simulink model "mpc_ttype_psm"  (R2026a)
settings: Solver=ode23tb  StopTime=param.sim.simlength  FixedStep=param.glb_time.tc  MaxStep=param.glb_time.tc
values from neighbouring files (symbols this model uses):
  param = struct()    [init_model.m]
libraries: fl_lib x25, nesl_utility x12, cstblocks_lti x6, lithium_ion_battery x1, dclink_for_three_levels x1, three_phase_three_level_ttype_inverter_ideal_switch_based_model x1, single_phase_pwm_modulator x1, threephase_inductor_lib x1, simple_flexible_shaft x1, permanent_magnet_synchronous_machine x1
(part 1 of 4)
settings Model: SimulationMode=accelerator  Creator=dbagn  LastModifiedBy=dbagn
settings SolverCC: NumberNewtonIterations=3.0  ZeroCrossControl=DisableAll  SolverResetMethod=Robust
settings SFSimCC: CustomCodeUndefinedFunction=ThrowError  DefaultCustomCodeDeterministicFunctions=All
settings SFSimCC: SimCustomHeaderCode=|
  | #include "rpi.h"
  | #include "mavgflt.h"
  | #include "mavgflt_simulink.h"
  | #include "mavgflts.h"
  | #include "mavgflts_simulink.h"
  | #include "dsmavgflt.h"
  | #include "dsmavgflt_simulink.h"
  | #include "bemf_obsv.h"
  | #include "bemf_obsv_simulink.h"
  | #include "bemf_obsv_load_est.h"
  | #include "bemf_obsv_load_est_simulink.h"
  | #include "dqvector_pi.h"
  | #include "dqvector_pi_simulink.h"
  | #include "sv_pwm_simulink.h"
  | #include "sv_pwm.h"
  | #include "first_harmonic_tracker.h"
  | #include "first_harmonic_tracker_simulink.h"
  | #include "dqpll_thyr.h"
  | #include "dqpll_thyr_simulink.h"
  | #include "dqpll_grid.h"
  | #include "dqpll_grid_simulink.h"
settings SFSimCC: SimUserSources=|
  | "rpi.c"
  | "mavgflt_simulink.c"
  | "mavgflt.c"
  | "mavgflts_simulink.c"
  | "mavgflts.c"
  | "dsmavgflt_simulink.c"
  | "dsmavgflt.c"
  | "bemf_obsv_simulink.c"
  | "bemf_obsv.c"
  | "bemf_obsv_load_est_simulink.c"
  | "bemf_obsv_load_est.c"
  | "dqvector_pi.c"
  | "dqvector_pi_simulink.c"
  | "sv_pwm_simulink.c"
  | "sv_pwm.c"
  | "first_harmonic_tracker_simulink.c"
  | "first_harmonic_tracker.c"
  | "dqpll_thyr_simulink.c"
  | "dqpll_thyr.c"
  | "dqpll_grid_simulink.c"
  | "dqpll_grid.c"
settings SFSimCC: SimUserIncludeDirs=|
  | include
  | src
settings SimscapeCC: SimscapeNominalValues="[{\"value\":\"1\",\"unit\":\"A\"},{\"value\":\"1\",\"unit\":\"bar\"},{\"value\":\"1\",\"unit\":\"cm^2\"},{\"value\":\"1\",\"unit\":\"cm^3/s\"},{\"value\":\"1\",\"unit\":\"kJ/kg\"},{\"value\":\"1\",\"unit\":\"kW\"},{\"value\":\"1\",\"unit\":\"l\"},{\"value\":\"1\",\"unit\":\"N\"},{\"value\":\"1\",\"unit\":\"N*m\"},{\"value\":\"1\",\"unit\":\"V\"}]"  SimscapeLogType=none  SimscapeLogDataHistory=5000.0

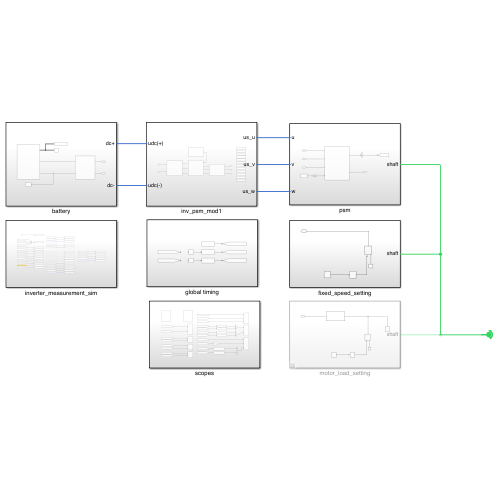
[thumbnail: Simulink's stored preview of the top-level diagram]
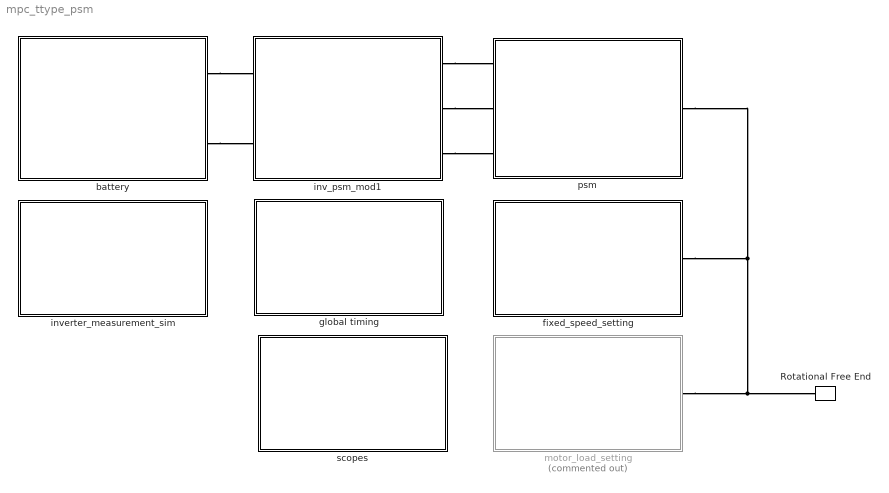
== system mpc_ttype_psm ==
  Rotational Free End : fl_lib/Mechanical/Rotational Elements/Rotational Free End  w_specify=off  w_priority=None  w=0 rad/s  w_nominal_specify=off  w_nominal_value=1  w_nominal_unit=rad/s
  battery : Subsystem
  fixed_speed_setting : Subsystem
  global timing : Subsystem
  inv_psm_mod1 : Subsystem
  inverter_measurement_sim : Subsystem
  motor_load_setting : Subsystem  Commented=on
  psm : Subsystem
  scopes : Subsystem
  connections:
  psm/RConn1 -- fixed_speed_setting/LConn1 -- motor_load_setting/LConn1 -- Rotational Free End/LConn1
  inv_psm_mod1/RConn2 -- psm/LConn2
  inv_psm_mod1/RConn1 -- psm/LConn1
  inv_psm_mod1/RConn3 -- psm/LConn3
  battery/RConn1 -- inv_psm_mod1/LConn1
  battery/RConn2 -- inv_psm_mod1/LConn2

== system mpc_ttype_psm/battery ==
  Solver Configuration : nesl_utility/Solver Configuration  PhysicalDomain=network_engine_domain  SubClassName=solver  LeftPortType=input  RightPortType=generic  Tones=[]  Harmonics=[]  SimulateNoise=off  Profile=off  UseLocalSampling=off  EnableSwitchedLinearOptims=on  FrequencyDomain=off  UseCCode=off  RelTol=0.001  AbsTol=0.001  MinStep=1e-09  ToWorkspace=off  RevertToSquareIcSolve=off  NumHomotopyIterations=100  PhasorMode=off  PhasorModeNumHarmonics=1  ConsistencySolver=NEWTON_FTOL  CanonicalOrdering=UNORDERED  OptimizeIntermediates=UNOPTIMIZED  IndexReductionMethod=DerivativeReplacement  DoDC=on  ResidualTolerance=1e-09  ConsistencyTolSource=GLOBAL  ConsistencyAbsTol=0.001  ConsistencyRelTol=0.001  ConsistencyTolFactor=0.001  UseLocalSolver=on  LocalSolverChoice=NE_BACKWARD_EULER_ADVANCER  ResolveIndetEquations=on  FunctionEvalNumThread=1  LocalSolverSampleTime=param.glb_time.tc  DoFixedCost=on  MaxNonlinIter=param.sim.nonlinear_iterations  MaxModeIter=2  ComputeImpulses=off  ImpulseIterations=2  LinearAlgebra=auto  LinearAlgebraNumThread=0  EquationFormulation=NE_TIME_EF  DelaysMemoryBudget=1024  AutomaticFiltering=on  FilteringTimeConstant=0.001  PartitionStorageMethod=AS_NEEDED  PartitionMemoryBudget=1024  PartitionMethod=ROBUST  MultibodyUseLocalSolver=off  MultibodyLocalSolverChoice=ODE1  MultibodyLocalSolverSampleTime=0.001
  To Workspace14 : ToWorkspace  VariableName=battery_data  SampleTime=param.glb_time.tc
      settings: MaxDataPoints=param.glb_time.Nc
  lithium ion battery : Scope
      settings: ActiveDisplayYMinimum=-146.3940131322023  ActiveDisplayYMaximum=1008.7733008785125  DataLoggingVariableName=ScopeData3
  lithium_ion_battery : lithium_ion_battery/lithium_ion_battery  Q=param.battery.pack_1.Q  number_of_cells=param.battery.pack_1.number_of_cells  E_1=param.battery.pack_1.E_1  E0=param.battery.pack_1.E0  E1=param.battery.pack_1.E1  E2=param.battery.pack_1.E2  E3=param.battery.pack_1.E3  Elog=param.battery.pack_1.Elog  R0=param.battery.pack_1.R0  R1=param.battery.pack_1.R1  C1=param.battery.pack_1.C1  M=param.battery.pack_1.M  alpha=param.battery.pack_1.alpha  soc_init=param.battery.pack_1.soc_init  ts_battery=param.glb_time.ts_dab  q1Kalman=param.battery.pack_1.q1Kalman  q2Kalman=param.battery.pack_1.q2Kalman  q3Kalman=param.battery.pack_1.q3Kalman  rKalman=param.battery.pack_1.rKalman  tc=param.glb_time.tc  enable_white_noise_m=0
  single_phase_ui_measure : Subsystem
  dc+ : PMIOPort  Side=Right
  dc- : PMIOPort  Port=2  Side=Right
  wires:
  lithium_ion_battery/1 -> To Workspace14/1, lithium ion battery/1
  connections:
  single_phase_ui_measure/LConn2 -- Solver Configuration/RConn1 -- lithium_ion_battery/RConn2
  single_phase_ui_measure/RConn1 -- dc+/RConn1
  lithium_ion_battery/RConn1 -- single_phase_ui_measure/LConn1
  dc-/RConn1 -- single_phase_ui_measure/RConn2

== system mpc_ttype_psm/fixed_speed_setting ==
  Ideal Angular Velocity Source : fl_lib/Mechanical/Mechanical Sources/Ideal Angular Velocity Source
  Mechanical Rotational Reference : fl_lib/Mechanical/Rotational Elements/Mechanical Rotational Reference
  PS Step1 : fl_lib/Physical Signals/Sources/PS Step  step_time=0.025 s  initial_value=0 rpm  final_value=param.load.rpm_sim rpm
  PS Transfer Function : fl_lib/Physical Signals/Linear Operators/PS Transfer Function  transfer_function_type=foundation.enum.transfer_function_type.lag  T=0.1 s  T1=2 s  T2=1 s  reset_method=foundation.enum.IntegratorResetSpec.None  initial_condition_spec=foundation.enum.IntegratorICSpec.Internal  y0=0 rpm
  shaft : PMIOPort  Side=Left
  connections:
  Mechanical Rotational Reference/LConn1 -- Ideal Angular Velocity Source/RConn2
  PS Step1/RConn1 -- PS Transfer Function/LConn1
  PS Transfer Function/RConn1 -- Ideal Angular Velocity Source/RConn1
  Ideal Angular Velocity Source/LConn1 -- shaft/RConn1

== system mpc_ttype_psm/global timing ==
  From9 : From  Commented=on  GotoTag=local_time_corr_afe1
  Unit Delay : UnitDelay  SampleTime=param.glb_time.tc
  Unit Delay1 : UnitDelay  SampleTime=param.glb_time.tc
  time_afe1 : Subsystem  mask{k=param.afe.behav.time_gain_module_1}
      mask prompts: k "Time Gain"
      mask Display:
      | disp('time-gen');
      | port_label('input', 1, 'crt');
      | port_label('output', 1, 'tout');
  time_afe3 : Subsystem  mask{k=1}
      mask prompts: k "Time Gain"
      mask Display:
      | disp('time-gen');
      | port_label('output', 1, 'tout');
  time_inv1 : Subsystem  mask{k=param.inv.behav.time_gain_module_2}
      mask prompts: k "Time Gain"
      mask Display:
      | disp('time-gen');
      | port_label('input', 1, 'crt');
      | port_label('output', 1, 'tout');
  tag scope: time_afe_module_1=global, time_inv_module_1=global, time_master=global
  wires:
  time_afe1/1(Out1) -> [time_afe_module_1]
  time_inv1/1(Out1) -> [time_inv_module_1]
  time_afe3/1(Out1) -> [time_master]
  Unit Delay/1 -> time_afe1/1(correction_time)
  Unit Delay1/1 -> time_inv1/1(correction_time)

== system mpc_ttype_psm/inv_psm_mod1 ==
  Goto Tag Visibility : GotoTagVisibility  GotoTag=vdc_pu
  Goto Tag Visibility1 : GotoTagVisibility  GotoTag=udc
  Goto Tag Visibility10 : GotoTagVisibility  GotoTag=udc1_pu
  Goto Tag Visibility11 : GotoTagVisibility  GotoTag=udc2_pu
  Goto Tag Visibility2 : GotoTagVisibility  GotoTag=udc1
  Goto Tag Visibility3 : GotoTagVisibility  GotoTag=udc2
  Goto Tag Visibility4 : GotoTagVisibility  GotoTag=np_current
  Goto Tag Visibility5 : GotoTagVisibility  GotoTag=udc_p_gnd
  Goto Tag Visibility6 : GotoTagVisibility  GotoTag=udc_n_gnd
  Goto Tag Visibility7 : GotoTagVisibility  GotoTag=udc_centertap_gnd
  Goto Tag Visibility8 : GotoTagVisibility  GotoTag=Cdc1_current
  Goto Tag Visibility9 : GotoTagVisibility  GotoTag=Cdc2_current
  dclink : Subsystem
  inverter : Subsystem
  inverter_ctrl : Subsystem
  inverter_output_filter : Subsystem
  us_u : PMIOPort  Side=Right
  us_v : PMIOPort  Port=2  Side=Right
  us_w : PMIOPort  Port=3  Side=Right
  udc(+) : PMIOPort  Port=4  Side=Left
  udc(-) : PMIOPort  Port=5  Side=Left
  wires:
  inverter_ctrl/1(cmd_gates) -> inverter/1(gate_cmds_uvw)
  connections:
  inverter_output_filter/LConn2 -- us_v/RConn1
  inverter_output_filter/LConn3 -- us_w/RConn1
  inverter_output_filter/LConn1 -- us_u/RConn1
  dclink/LConn1 -- udc(+)/RConn1
  dclink/LConn2 -- udc(-)/RConn1
  inverter/RConn2 -- dclink/RConn2
  inverter/RConn1 -- dclink/RConn1
  inverter/RConn3 -- dclink/RConn3
  inverter_output_filter/RConn3 -- inverter/LConn3
  inverter_output_filter/RConn2 -- inverter/LConn2
  inverter_output_filter/RConn1 -- inverter/LConn1

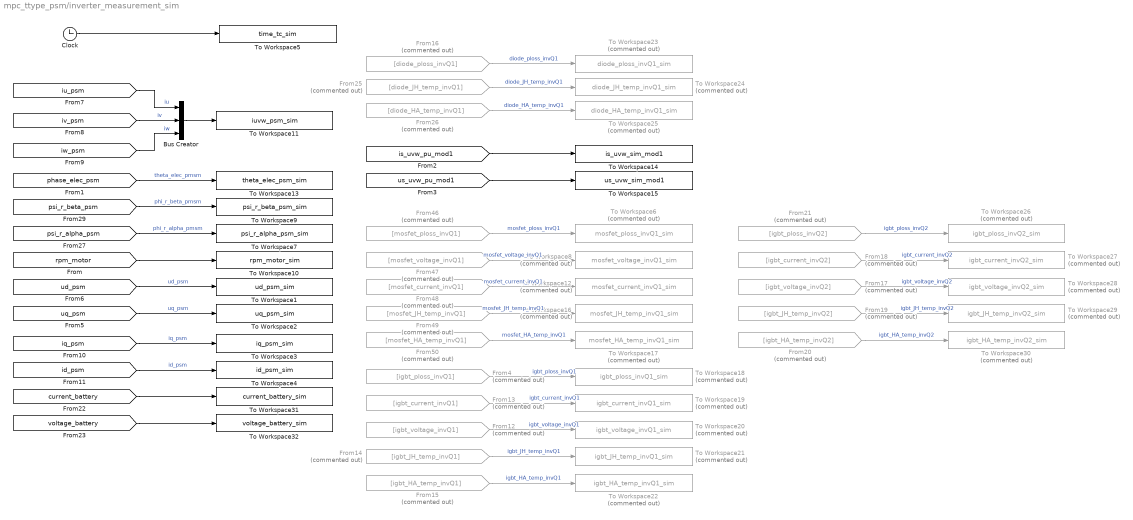
== system mpc_ttype_psm/inverter_measurement_sim ==
  Bus Creator : BusCreator  Inputs=3
  Clock : Clock
  From12 : From  Commented=on  GotoTag=igbt_voltage_invQ1
  From13 : From  Commented=on  GotoTag=igbt_current_invQ1
  From14 : From  Commented=on  GotoTag=igbt_JH_temp_invQ1
  From15 : From  Commented=on  GotoTag=igbt_HA_temp_invQ1
  From16 : From  Commented=on  GotoTag=diode_ploss_invQ1
  From17 : From  Commented=on  GotoTag=igbt_voltage_invQ2
  From18 : From  Commented=on  GotoTag=igbt_current_invQ2
  From19 : From  Commented=on  GotoTag=igbt_JH_temp_invQ2
  From20 : From  Commented=on  GotoTag=igbt_HA_temp_invQ2
  From21 : From  Commented=on  GotoTag=igbt_ploss_invQ2
  From25 : From  Commented=on  GotoTag=diode_JH_temp_invQ1
  From26 : From  Commented=on  GotoTag=diode_HA_temp_invQ1
  From4 : From  Commented=on  GotoTag=igbt_ploss_invQ1
  From46 : From  Commented=on  GotoTag=mosfet_ploss_invQ1
  From47 : From  Commented=on  GotoTag=mosfet_voltage_invQ1
  From48 : From  Commented=on  GotoTag=mosfet_current_invQ1
  From49 : From  Commented=on  GotoTag=mosfet_JH_temp_invQ1
  From50 : From  Commented=on  GotoTag=mosfet_HA_temp_invQ1
  To Workspace1 : ToWorkspace  VariableName=ud_psm_sim  SampleTime=param.glb_time.tc
      settings: MaxDataPoints=param.glb_time.Nc  Save2DSignal=2-D array (concatenate along first dimension)
  To Workspace10 : ToWorkspace  VariableName=rpm_motor_sim  SampleTime=param.glb_time.tc
      settings: MaxDataPoints=param.glb_time.Nc  Save2DSignal=2-D array (concatenate along first dimension)
  To Workspace11 : ToWorkspace  VariableName=iuvw_psm_sim  SampleTime=param.glb_time.tc
      settings: MaxDataPoints=param.glb_time.Nc  Save2DSignal=2-D array (concatenate along first dimension)
  To Workspace12 : ToWorkspace  Commented=on  VariableName=mosfet_current_invQ1_sim  SampleTime=param.glb_time.tc
      settings: MaxDataPoints=param.glb_time.Nc  Save2DSignal=2-D array (concatenate along first dimension)
  To Workspace13 : ToWorkspace  VariableName=theta_elec_psm_sim  SampleTime=param.glb_time.tc
      settings: MaxDataPoints=param.glb_time.Nc  Save2DSignal=2-D array (concatenate along first dimension)
  To Workspace14 : ToWorkspace  VariableName=is_uvw_sim_mod1  SampleTime=param.glb_time.tc
      settings: MaxDataPoints=param.glb_time.Nc  Save2DSignal=2-D array (concatenate along first dimension)
  To Workspace15 : ToWorkspace  VariableName=us_uvw_sim_mod1  SampleTime=param.glb_time.tc
      settings: MaxDataPoints=param.glb_time.Nc  Save2DSignal=2-D array (concatenate along first dimension)
  To Workspace16 : ToWorkspace  Commented=on  VariableName=mosfet_JH_temp_invQ1_sim  SampleTime=param.glb_time.tc
      settings: MaxDataPoints=param.glb_time.Nc  Save2DSignal=2-D array (concatenate along first dimension)
  To Workspace17 : ToWorkspace  Commented=on  VariableName=mosfet_HA_temp_invQ1_sim  SampleTime=param.glb_time.tc
      settings: MaxDataPoints=param.glb_time.Nc  Save2DSignal=2-D array (concatenate along first dimension)
  To Workspace18 : ToWorkspace  Commented=on  VariableName=igbt_ploss_invQ1_sim  SampleTime=param.glb_time.tc
      settings: MaxDataPoints=param.glb_time.Nc  Save2DSignal=2-D array (concatenate along first dimension)
  To Workspace19 : ToWorkspace  Commented=on  VariableName=igbt_current_invQ1_sim  SampleTime=param.glb_time.tc
      settings: MaxDataPoints=param.glb_time.Nc  Save2DSignal=2-D array (concatenate along first dimension)
  To Workspace2 : ToWorkspace  VariableName=uq_psm_sim  SampleTime=param.glb_time.tc
      settings: MaxDataPoints=param.glb_time.Nc  Save2DSignal=2-D array (concatenate along first dimension)
  To Workspace20 : ToWorkspace  Commented=on  VariableName=igbt_voltage_invQ1_sim  SampleTime=param.glb_time.tc
      settings: MaxDataPoints=param.glb_time.Nc  Save2DSignal=2-D array (concatenate along first dimension)
  To Workspace21 : ToWorkspace  Commented=on  VariableName=igbt_JH_temp_invQ1_sim  SampleTime=param.glb_time.tc
      settings: MaxDataPoints=param.glb_time.Nc  Save2DSignal=2-D array (concatenate along first dimension)
  To Workspace22 : ToWorkspace  Commented=on  VariableName=igbt_HA_temp_invQ1_sim  SampleTime=param.glb_time.tc
      settings: MaxDataPoints=param.glb_time.Nc  Save2DSignal=2-D array (concatenate along first dimension)
  To Workspace23 : ToWorkspace  Commented=on  VariableName=diode_ploss_invQ1_sim  SampleTime=param.glb_time.tc
      settings: MaxDataPoints=param.glb_time.Nc
  To Workspace24 : ToWorkspace  Commented=on  VariableName=diode_JH_temp_invQ1_sim  SampleTime=param.glb_time.tc
      settings: MaxDataPoints=param.glb_time.Nc
  To Workspace25 : ToWorkspace  Commented=on  VariableName=diode_HA_temp_invQ1_sim  SampleTime=param.glb_time.tc
      settings: MaxDataPoints=param.glb_time.Nc
  To Workspace26 : ToWorkspace  Commented=on  VariableName=igbt_ploss_invQ2_sim  SampleTime=param.glb_time.tc
      settings: MaxDataPoints=param.glb_time.Nc  Save2DSignal=2-D array (concatenate along first dimension)
  To Workspace27 : ToWorkspace  Commented=on  VariableName=igbt_current_invQ2_sim  SampleTime=param.glb_time.tc
      settings: MaxDataPoints=param.glb_time.Nc  Save2DSignal=2-D array (concatenate along first dimension)
  To Workspace28 : ToWorkspace  Commented=on  VariableName=igbt_voltage_invQ2_sim  SampleTime=param.glb_time.tc
      settings: MaxDataPoints=param.glb_time.Nc  Save2DSignal=2-D array (concatenate along first dimension)
  To Workspace29 : ToWorkspace  Commented=on  VariableName=igbt_JH_temp_invQ2_sim  SampleTime=param.glb_time.tc
      settings: MaxDataPoints=param.glb_time.Nc  Save2DSignal=2-D array (concatenate along first dimension)
  To Workspace3 : ToWorkspace  VariableName=iq_psm_sim  SampleTime=param.glb_time.tc
      settings: MaxDataPoints=param.glb_time.Nc  Save2DSignal=2-D array (concatenate along first dimension)
  To Workspace30 : ToWorkspace  Commented=on  VariableName=igbt_HA_temp_invQ2_sim  SampleTime=param.glb_time.tc
      settings: MaxDataPoints=param.glb_time.Nc  Save2DSignal=2-D array (concatenate along first dimension)
  To Workspace31 : ToWorkspace  VariableName=current_battery_sim  SampleTime=param.glb_time.tc
      settings: MaxDataPoints=param.glb_time.Nc  Save2DSignal=2-D array (concatenate along first dimension)
  To Workspace32 : ToWorkspace  VariableName=voltage_battery_sim  SampleTime=param.glb_time.tc
      settings: MaxDataPoints=param.glb_time.Nc  Save2DSignal=2-D array (concatenate along first dimension)
  To Workspace4 : ToWorkspace  VariableName=id_psm_sim  SampleTime=param.glb_time.tc
      settings: MaxDataPoints=param.glb_time.Nc  Save2DSignal=2-D array (concatenate along first dimension)
  To Workspace5 : ToWorkspace  VariableName=time_tc_sim  SampleTime=param.glb_time.tc
      settings: MaxDataPoints=param.glb_time.Nc  Save2DSignal=2-D array (concatenate along first dimension)
  To Workspace6 : ToWorkspace  Commented=on  VariableName=mosfet_ploss_invQ1_sim  SampleTime=param.glb_time.tc
      settings: MaxDataPoints=param.glb_time.Nc  Save2DSignal=2-D array (concatenate along first dimension)
  To Workspace7 : ToWorkspace  VariableName=psi_r_alpha_psm_sim  SampleTime=param.glb_time.tc
      settings: MaxDataPoints=param.glb_time.Nc  Save2DSignal=2-D array (concatenate along first dimension)
  To Workspace8 : ToWorkspace  Commented=on  VariableName=mosfet_voltage_invQ1_sim  SampleTime=param.glb_time.tc
      settings: MaxDataPoints=param.glb_time.Nc  Save2DSignal=2-D array (concatenate along first dimension)
  To Workspace9 : ToWorkspace  VariableName=psi_r_beta_psm_sim  SampleTime=param.glb_time.tc
      settings: MaxDataPoints=param.glb_time.Nc  Save2DSignal=2-D array (concatenate along first dimension)
  wires:
  [psi_r_alpha_psm] -> To Workspace7/1  "phi_r_alpha_pmsm"
  [psi_r_beta_psm] -> To Workspace9/1  "phi_r_beta_pmsm"
  [rpm_motor] -> To Workspace10/1
  [iv_psm] -> Bus Creator/2  "iv"
  [iw_psm] -> Bus Creator/3  "iw"
  [iu_psm] -> Bus Creator/1  "iu"
  Bus Creator/1 -> To Workspace11/1
  [phase_elec_psm] -> To Workspace13/1  "theta_elec_pmsm"
  [ud_psm] -> To Workspace1/1  "ud_psm"
  [uq_psm] -> To Workspace2/1  "uq_psm"
  [iq_psm] -> To Workspace3/1  "iq_psm"
  [id_psm] -> To Workspace4/1  "id_psm"
  Clock/1 -> To Workspace5/1
  From46/1 -> To Workspace6/1  "mosfet_ploss_invQ1"
  From49/1 -> To Workspace16/1  "mosfet_JH_temp_invQ1"
  From50/1 -> To Workspace17/1  "mosfet_HA_temp_invQ1"
  [is_uvw_pu_mod1] -> To Workspace14/1
  [us_uvw_pu_mod1] -> To Workspace15/1
  From47/1 -> To Workspace8/1  "mosfet_voltage_invQ1"
  From48/1 -> To Workspace12/1  "mosfet_current_invQ1"
  From4/1 -> To Workspace18/1  "igbt_ploss_invQ1"
  From13/1 -> To Workspace19/1  "igbt_current_invQ1"
  From12/1 -> To Workspace20/1  "igbt_voltage_invQ1"
  From14/1 -> To Workspace21/1  "igbt_JH_temp_invQ1"
  From15/1 -> To Workspace22/1  "igbt_HA_temp_invQ1"
  From16/1 -> To Workspace23/1  "diode_ploss_invQ1"
  From25/1 -> To Workspace24/1  "diode_JH_temp_invQ1"
  From26/1 -> To Workspace25/1  "diode_HA_temp_invQ1"
  From20/1 -> To Workspace30/1  "igbt_HA_temp_invQ2"
  From19/1 -> To Workspace29/1  "igbt_JH_temp_invQ2"
  From17/1 -> To Workspace28/1  "igbt_voltage_invQ2"
  From18/1 -> To Workspace27/1  "igbt_current_invQ2"
  From21/1 -> To Workspace26/1  "igbt_ploss_invQ2"
  [current_battery] -> To Workspace31/1
  [voltage_battery] -> To Workspace32/1

== system mpc_ttype_psm/motor_load_setting ==
  Ideal Torque Source : fl_lib/Mechanical/Mechanical Sources/Ideal Torque Source
  Inertia : fl_lib/Mechanical/Rotational Elements/Inertia  inertia=param.load.external_load_inertia kg*m^2  num_ports=foundation.enum.numPorts2.one  w_specify=off  w_priority=High  w=0 rad/s  w_nominal_specify=off  w_nominal_value=1  w_nominal_unit=rad/s  t_specify=off  t_priority=None  t=0 N*m  t_nominal_specify=off  t_nominal_value=1  t_nominal_unit=N*m
  Mechanical Rotational Reference : fl_lib/Mechanical/Rotational Elements/Mechanical Rotational Reference
  PS Step : fl_lib/Physical Signals/Sources/PS Step  step_time=param.sim.load_step_time s  initial_value=1 N*m  final_value=1 N*m
  PS Transfer Function : fl_lib/Physical Signals/Linear Operators/PS Transfer Function  transfer_function_type=foundation.enum.transfer_function_type.lag  T=1 s  T1=2 s  T2=1 s  reset_method=foundation.enum.IntegratorResetSpec.None  initial_condition_spec=foundation.enum.IntegratorICSpec.Internal  y0=0 N*m
  flexible_shaft : simple_flexible_shaft/flexible_shaft  b1=1  b2=1  J1=1  J2=1  b_displacement=1  k_displacement=1e5
  shaft : PMIOPort  Side=Left
  connections:
  Ideal Torque Source/LConn1 -- flexible_shaft/RConn1 -- Inertia/LConn1
  Ideal Torque Source/RConn2 -- Mechanical Rotational Reference/LConn1
  PS Transfer Function/RConn1 -- Ideal Torque Source/RConn1
  PS Step/RConn1 -- PS Transfer Function/LConn1
  flexible_shaft/LConn1 -- shaft/RConn1

== system mpc_ttype_psm/psm ==
  Bus Selector1 : BusSelector  OutputSignals=omega_mech (rpm)
  Constant : Constant  Value=param.psm.machine.psi_m
  Simulink-PS Converter3 : nesl_utility/Simulink-PS Converter  PhysicalDomain=network_engine_domain  SubClassName=ps_input  LeftPortType=input  RightPortType=output  PseudoPeriodic=off  Frequencies=[]  NoiseDistribution=none  NoiseParameters=[]  Unit=V*s  AffineConversion=on  FilteringAndDerivatives=provide  SimscapeFilterOrder=1  InputFilterTimeConstant=0.001  UdotUserProvided=0
  synchronous_motor : Subsystem
  u : PMIOPort  Side=Left
  v : PMIOPort  Port=2  Side=Left
  w : PMIOPort  Port=3  Side=Left
  shaft : PMIOPort  Port=4  Side=Right
  tag scope: rpm_motor=global
  wires:
  synchronous_motor/1(motor_data) -> Bus Selector1/1
  Bus Selector1/1 -> [rpm_motor]  "<omega_mech (rpm)>"
  Constant/1 -> Simulink-PS Converter3/1
  connections:
  synchronous_motor/LConn1 -- u/RConn1
  Simulink-PS Converter3/RConn1 -- synchronous_motor/LConn4
  synchronous_motor/LConn3 -- w/RConn1
  synchronous_motor/LConn2 -- v/RConn1
  shaft/RConn1 -- synchronous_motor/RConn1

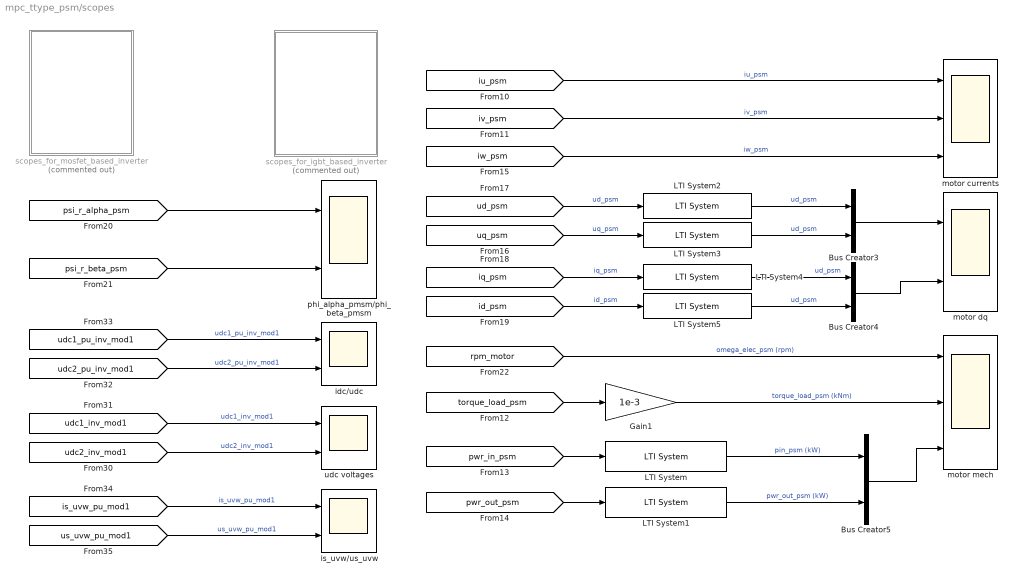
== system mpc_ttype_psm/scopes ==
  Bus Creator3 : BusCreator  Inputs=2
  Bus Creator4 : BusCreator  Inputs=2
  Bus Creator5 : BusCreator  Inputs=2
  Gain1 : Gain  Gain=1e-3
  LTI System{,1..5} (6 alike) : cstblocks_lti/LTI System  sys=param.ctrl.filters.inv.SOF_50Hz.ss_c  IC=[]  PadeOrder=0
  idc/udc : Scope  NumInputPorts=2
      settings: SampleTime=param.glb_time.tc  ActiveDisplayYMinimum=-429.79232670429462  ActiveDisplayYMaximum=486.89839586541632  DataLoggingVariableName=ScopeData23
  is_uvw/us_uvw : Scope  NumInputPorts=2
      settings: SampleTime=param.glb_time.tc  ActiveDisplayYMinimum=-4.0901889520524559  ActiveDisplayYMaximum=4.1379165768312332  DataLoggingVariableName=ScopeData25
  motor currents : Scope  NumInputPorts=3
      settings: SampleTime=param.glb_time.tc  ActiveDisplayYMinimum=-474.88865629966676  ActiveDisplayYMaximum=470.37643994604952  DataLoggingVariableName=ScopeData17
  motor dq : Scope  NumInputPorts=2
      settings: SampleTime=param.glb_time.tc  ActiveDisplayYMinimum=-441.73115786149134  ActiveDisplayYMaximum=53.6844226840948  DataLoggingVariableName=ScopeData18
  motor mech : Scope  NumInputPorts=3
      settings: SampleTime=param.glb_time.tc  ActiveDisplayYMinimum=15.405374824722539  ActiveDisplayYMaximum=15.477183050334578  DataLoggingVariableName=ScopeData11
  phi_alpha_pmsm/phi_beta_pmsm : Scope  NumInputPorts=2
      settings: SampleTime=param.glb_time.tc  ActiveDisplayYMinimum=-4.800821748013445  ActiveDisplayYMaximum=4.8008423854253959  DataLoggingVariableName=ScopeData19
  scopes_for_igbt_based_inverter : Subsystem  Commented=on
  scopes_for_mosfet_based_inverter : Subsystem  Commented=on
  udc voltages : Scope  NumInputPorts=2
      settings: SampleTime=param.glb_time.tc  ActiveDisplayYMinimum=585.40162224007008  ActiveDisplayYMaximum=587.2891594036563  DataLoggingVariableName=ScopeData24
  wires:
  [torque_load_psm] -> Gain1/1
  [pwr_out_psm] -> LTI System1/1
  Bus Creator4/1 -> motor dq/2
  LTI System/1 -> Bus Creator5/1  "pin_psm (kW)"
  LTI System1/1 -> Bus Creator5/2  "pwr_out_psm (kW)"
  [iw_psm] -> motor currents/3  "iw_psm"
  Gain1/1 -> motor mech/2  "torque_load_psm (kNm)"
  [id_psm] -> LTI System5/1  "id_psm"
  [psi_r_alpha_psm] -> phi_alpha_pmsm/phi_beta_pmsm/1
  [iv_psm] -> motor currents/2  "iv_psm"
  Bus Creator3/1 -> motor dq/1
  [uq_psm] -> LTI System3/1  "uq_psm"
  [iu_psm] -> motor currents/1  "iu_psm"
  Bus Creator5/1 -> motor mech/3
  [ud_psm] -> LTI System2/1  "ud_psm"
  [iq_psm] -> LTI System4/1  "iq_psm"
  [rpm_motor] -> motor mech/1  "omega_elec_psm (rpm)"
  [pwr_in_psm] -> LTI System/1
  [psi_r_beta_psm] -> phi_alpha_pmsm/phi_beta_pmsm/2
  [udc1_inv_mod1] -> udc voltages/1  "udc1_inv_mod1"
  [udc1_pu_inv_mod1] -> idc/udc/1  "udc1_pu_inv_mod1"
  [udc2_pu_inv_mod1] -> idc/udc/2  "udc2_pu_inv_mod1"
  [udc2_inv_mod1] -> udc voltages/2  "udc2_inv_mod1"
  [is_uvw_pu_mod1] -> is_uvw/us_uvw/1  "is_uvw_pu_mod1"
  [us_uvw_pu_mod1] -> is_uvw/us_uvw/2  "us_uvw_pu_mod1"
  LTI System2/1 -> Bus Creator3/1  "ud_psm"
  LTI System3/1 -> Bus Creator3/2  "ud_psm"
  LTI System4/1 -> Bus Creator4/1  "ud_psm"
  LTI System5/1 -> Bus Creator4/2  "ud_psm"

== system mpc_ttype_psm/battery/single_phase_ui_measure ==
  Bus Creator : BusCreator  Inputs=2
  Current Sensor : fl_lib/Electrical/Electrical Sensors/Current Sensor
  Selector : Selector  InputPortWidth=2  IndexOptions=Index vector (dialog)  Indices=2  OutputSizes=1
  Selector1 : Selector  InputPortWidth=2  IndexOptions=Index vector (dialog)  Indices=1  OutputSizes=1
  Voltage Sensor : fl_lib/Electrical/Electrical Sensors/Voltage Sensor
  dab input modA : Scope  NumInputPorts=2
      settings: SampleTime=param.glb_time.tc  ActiveDisplayYMinimum=-45.035005749774236  ActiveDisplayYMaximum=-4.6312000589885987  DataLoggingVariableName=ScopeData7
  iph : nesl_utility/PS-Simulink Converter  PhysicalDomain=network_engine_domain  SubClassName=ps_output  LeftPortType=input  RightPortType=output  PseudoPeriodic=off  Frequencies=[]  VectorFormat=1-D array  Unit=A  AffineConversion=off
  uph : nesl_utility/PS-Simulink Converter  PhysicalDomain=network_engine_domain  SubClassName=ps_output  LeftPortType=input  RightPortType=output  PseudoPeriodic=off  Frequencies=[]  VectorFormat=1-D array  Unit=V  AffineConversion=off
  Udc(+) : PMIOPort  Side=Left
  udc(+) : PMIOPort  Port=2  Side=Right
  Udc(-) : PMIOPort  Port=3  Side=Left
  udc(-) : PMIOPort  Port=4  Side=Right
  tag scope: current_battery=global, voltage_battery=global
  wires:
  Bus Creator/1 -> Selector/1, Selector1/1  "ui_data"
  iph/1 -> Bus Creator/1  "iph"
  uph/1 -> Bus Creator/2  "uph"
  Selector1/1 -> dab input modA/1, [current_battery]  "current_battery"
  Selector/1 -> dab input modA/2, [voltage_battery]  "voltage_battery"
  connections:
  iph/LConn1 -- Current Sensor/RConn1
  Voltage Sensor/LConn1 -- Current Sensor/LConn1 -- Udc(+)/RConn1
  Current Sensor/RConn2 -- udc(+)/RConn1
  Voltage Sensor/RConn1 -- uph/LConn1
  Voltage Sensor/RConn2 -- Udc(-)/RConn1 -- udc(-)/RConn1

== system mpc_ttype_psm/global timing/time_afe1 ==
  correction_time : Inport
  Constant : Constant
  Gain : Gain  Gain=k
  Product : Product
  Sum : Sum  Inputs=|++
  time_1 : Clock
  Out1 : Outport
  wires:
  time_1/1 -> Gain/1
  Gain/1 -> Product/1
  Product/1 -> Out1/1
  correction_time/1 -> Sum/1
  Sum/1 -> Product/2
  Constant/1 -> Sum/2

== system mpc_ttype_psm/global timing/time_afe3 ==
  Gain : Gain  Gain=k
  time_1 : Clock
  Out1 : Outport
  wires:
  Gain/1 -> Out1/1
  time_1/1 -> Gain/1

== system mpc_ttype_psm/global timing/time_inv1 ==
  correction_time : Inport
  Constant : Constant
  Gain : Gain  Gain=k
  Product : Product
  Sum : Sum  Inputs=|++
  time_1 : Clock
  Out1 : Outport
  wires:
  time_1/1 -> Gain/1
  Gain/1 -> Product/1
  Product/1 -> Out1/1
  correction_time/1 -> Sum/1
  Constant/1 -> Sum/2
  Sum/1 -> Product/2

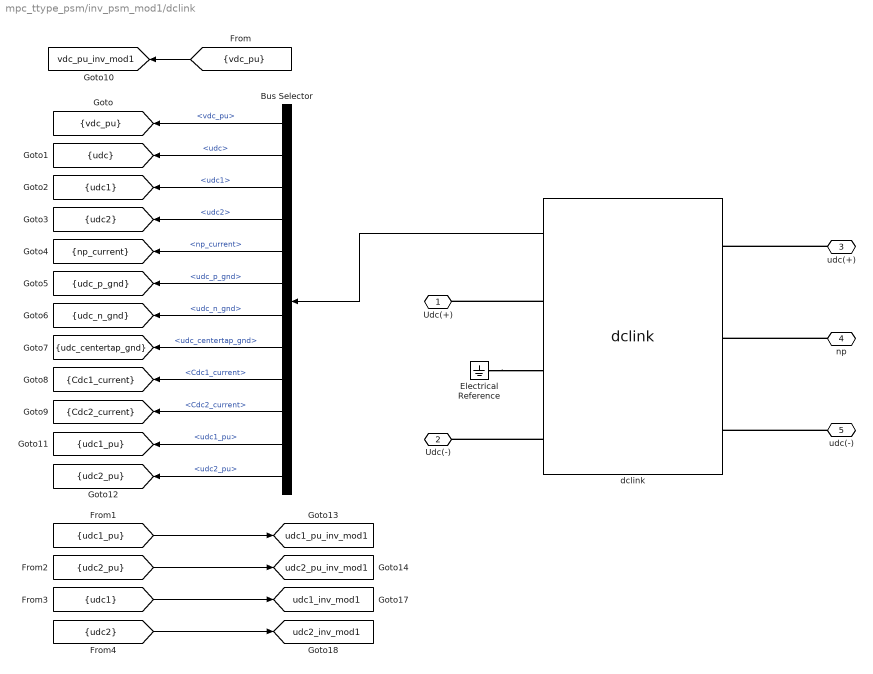
== system mpc_ttype_psm/inv_psm_mod1/dclink ==
  Bus Selector : BusSelector  OutputSignals=vdc_pu,udc,udc1,udc2,np_current,udc_p_gnd,udc_n_gnd,udc_centertap_gnd,Cdc1_current,Cdc2_current,udc1_pu,udc2_pu
  Electrical Reference : fl_lib/Electrical/Electrical Elements/Electrical Reference
  dclink : dclink_for_three_levels/dclink  Cdc1_m=param.inv.hw.CFi1  Cdc2_m=param.inv.hw.CFi2  Rudc_measure=param.inv.hw.Rudc_measure  Vdc_scale=param.inv.hw.udc_nom  Vdc1_m_init=param.inv.hw.udc_nom/2  Vdc2_m_init=param.inv.hw.udc_nom/2
  Udc(+) : PMIOPort  Side=Left
  Udc(-) : PMIOPort  Port=2  Side=Left
  udc(+) : PMIOPort  Port=3  Side=Right
  np : PMIOPort  Port=4  Side=Right
  udc(-) : PMIOPort  Port=5  Side=Right
  tag scope: Cdc1_current=scoped, Cdc2_current=scoped, np_current=scoped, udc1=scoped, udc1_inv_mod1=global, udc1_pu=scoped, udc1_pu_inv_mod1=global, udc2=scoped, udc2_inv_mod1=global, udc2_pu=scoped, udc2_pu_inv_mod1=global, udc=scoped, udc_centertap_gnd=scoped, udc_n_gnd=scoped, udc_p_gnd=scoped, vdc_pu=scoped, vdc_pu_inv_mod1=global
  wires:
  Bus Selector/6 -> [udc_p_gnd]  "<udc_p_gnd>"
  Bus Selector/8 -> [udc_centertap_gnd]  "<udc_centertap_gnd>"
  Bus Selector/2 -> [udc]  "<udc>"
  Bus Selector/7 -> [udc_n_gnd]  "<udc_n_gnd>"
  dclink/1 -> Bus Selector/1
  Bus Selector/4 -> [udc2]  "<udc2>"
  Bus Selector/9 -> [Cdc1_current]  "<Cdc1_current>"
  Bus Selector/5 -> [np_current]  "<np_current>"
  Bus Selector/3 -> [udc1]  "<udc1>"
  Bus Selector/10 -> [Cdc2_current]  "<Cdc2_current>"
  [vdc_pu] -> [vdc_pu_inv_mod1]
  Bus Selector/12 -> [udc2_pu]  "<udc2_pu>"
  Bus Selector/11 -> [udc1_pu]  "<udc1_pu>"
  [udc1_pu] -> [udc1_pu_inv_mod1]
  [udc2_pu] -> [udc2_pu_inv_mod1]
  [udc2] -> [udc2_inv_mod1]
  [udc1] -> [udc1_inv_mod1]
  Bus Selector/1 -> [vdc_pu]  "<vdc_pu>"
  connections:
  dclink/RConn3 -- Udc(-)/RConn1
  dclink/RConn1 -- Udc(+)/RConn1
  udc(+)/RConn1 -- dclink/LConn1
  np/RConn1 -- dclink/LConn2
  udc(-)/RConn1 -- dclink/LConn3
  Electrical Reference/LConn1 -- dclink/RConn2

== system mpc_ttype_psm/inv_psm_mod1/inverter ==
  gate_cmds_uvw : Inport
  Bus Creator : BusCreator  Inputs=2
  Current Sensor : fl_lib/Electrical/Electrical Sensors/Current Sensor
  PS-Simulink Converter1 : nesl_utility/PS-Simulink Converter  PhysicalDomain=network_engine_domain  SubClassName=ps_output  LeftPortType=input  RightPortType=output  PseudoPeriodic=off  Frequencies=[]  VectorFormat=1-D array  Unit=A  AffineConversion=on
  PS-Simulink Converter4 : nesl_utility/PS-Simulink Converter  PhysicalDomain=network_engine_domain  SubClassName=ps_output  LeftPortType=input  RightPortType=output  PseudoPeriodic=off  Frequencies=[]  VectorFormat=1-D array  Unit=V  AffineConversion=on
  To Workspace : ToWorkspace  VariableName=idc_sim_mod1  SampleTime=param.glb_time.tc
      settings: MaxDataPoints=param.glb_time.Nc
  To Workspace1 : ToWorkspace  VariableName=udc_sim_mod1  SampleTime=param.glb_time.tc
      settings: MaxDataPoints=param.glb_time.Nc
  Transfer Fcn : TransferFcn  Denominator=[1e-2 1]
  Voltage Sensor : fl_lib/Electrical/Electrical Sensors/Voltage Sensor
  deadtime_generator_for_ttype : Subsystem
  idc/udc : Scope  NumInputPorts=2
      settings: SampleTime=param.glb_time.tc  ActiveDisplayYMinimum=-35.22322330009689  ActiveDisplayYMaximum=317.00900970087207  DataLoggingVariableName=ScopeData8
  ideal_switch_based_three_level_inverter_ttype : three_phase_three_level_ttype_inverter_ideal_switch_based_model/ideal_switch_based_three_level_inverter_ttype  Vth=5.5  Ron=1.5e-3  Vdon_diode=2  Rdon_diode=0.15e-3  Csnubber=10e-9  Rsnubber=2200
  timer : Subsystem  mask{f=param.glb_time.fPWM_INV, m_up=0.98, m_low=0.02, dead_time=param.glb_time.dead_time_INV, pos_cmd_gate=15, neg_cmd_gate=-10, polarity=1, tc=param.glb_time.tc, double_sampling=param.glb_time.TRGO_INV_double_update}
      mask prompts: f "Frequency (Hz)"; m_up "Max Input Modulation Value"; m_low "Min Input Modulation Value"; dead_time "Dead Time (s)"; pos_cmd_gate "Positive Gate Voltage (V)"; neg_cmd_gate "Negative Gate Voltage (V)"; polarity "Polarity (pu)"; tc "Sampling time"
  udc_scope : Scope  NumInputPorts=3
      settings: ActiveDisplayYMinimum=0.97742270953395249  ActiveDisplayYMaximum=0.98060545699905033  DataLoggingVariableName=ScopeData6
  Udc(+) : PMIOPort  Side=Right
  np : PMIOPort  Port=2  Side=Right
  Udc(-) : PMIOPort  Port=3  Side=Right
  us_u : PMIOPort  Port=4  Side=Left
  us_v : PMIOPort  Port=5  Side=Left
  us_w : PMIOPort  Port=6  Side=Left
  tag scope: TRGO_inv_module_1=global
  wires:
  PS-Simulink Converter4/1 -> To Workspace1/1, idc/udc/2  "udc"
  PS-Simulink Converter1/1 -> Transfer Fcn/1  "idc"
  Transfer Fcn/1 -> idc/udc/1, To Workspace/1  "idc_flt"
  [vdc_pu] -> udc_scope/2  "udc_pu"
  [udc] -> udc_scope/1  "udc"
  [time_inv_module_1] -> timer/1(time_source)
  timer/1(TRGO) -> [TRGO_inv_module_1]
  gate_cmds_uvw/1 -> deadtime_generator_for_ttype/1(gate_cmds_in)
  deadtime_generator_for_ttype/1(gate_cmds_out) -> ideal_switch_based_three_level_inverter_ttype/1
  [udc1] -> Bus Creator/1  "udc_1"
  [udc2] -> Bus Creator/2  "udc_2"
  Bus Creator/1 -> udc_scope/3
  connections:
  PS-Simulink Converter4/LConn1 -- Voltage Sensor/RConn1
  ideal_switch_based_three_level_inverter_ttype/LConn1 -- us_u/RConn1
  ideal_switch_based_three_level_inverter_ttype/LConn2 -- us_v/RConn1
  ideal_switch_based_three_level_inverter_ttype/LConn3 -- us_w/RConn1
  Voltage Sensor/RConn2 -- ideal_switch_based_three_level_inverter_ttype/RConn3 -- Udc(-)/RConn1
  Current Sensor/LConn1 -- Udc(+)/RConn1
  Voltage Sensor/LConn1 -- ideal_switch_based_three_level_inverter_ttype/RConn1 -- Current Sensor/RConn2
  PS-Simulink Converter1/LConn1 -- Current Sensor/RConn1
  np/RConn1 -- ideal_switch_based_three_level_inverter_ttype/RConn2

== system mpc_ttype_psm/inv_psm_mod1/inverter_ctrl ==
  inverter_control : Subsystem
  cmd_gates : Outport
  tag scope: local_time_corr_inv1=global, master_torque_ref=global
  wires:
  [is_uvw_pu_mod1] -> inverter_control/1(is_uvw)
  [TRGO_inv_module_1] -> inverter_control/Trigger
  inverter_control/1(cmd_gates) -> cmd_gates/1
  [time_inv_module_1] -> inverter_control/4(local_time)
  [time_master] -> inverter_control/5(master_time)
  inverter_control/2(local_time_corr) -> [local_time_corr_inv1]
  inverter_control/3(master_torque_ref) -> [master_torque_ref]
  [phase_elec_psm] -> inverter_control/6(theta_elec_psm)
  [omega_elec_psm] -> inverter_control/7(omega_elec_psm)
  [udc1_pu] -> inverter_control/2(udc1_pu)  "udc1_pu"
  [udc2_pu] -> inverter_control/3(udc2_pu)  "udc2_pu"

== system mpc_ttype_psm/inv_psm_mod1/inverter_output_filter ==
  Inductor : fl_lib/Electrical/Electrical Elements/Inductor  l=1e-6 H  r=0 Ohm  g=1e-9 1/Ohm  i_specify=off  i_priority=None  i=0 A  i_nominal_specify=off  i_nominal_value=1  i_nominal_unit=A  v_specify=off  v_priority=None  v=0 V  v_nominal_specify=off  v_nominal_value=1  v_nominal_unit=V  i_L_specify=off  i_L_priority=High  i_L=0 A  i_L_nominal_specify=off  i_L_nominal_value=1  i_L_nominal_unit=A
  Inductor1 : fl_lib/Electrical/Electrical Elements/Inductor  l=1e-6 H  r=0 Ohm  g=1e-9 1/Ohm  i_specify=off  i_priority=None  i=0 A  i_nominal_specify=off  i_nominal_value=1  i_nominal_unit=A  v_specify=off  v_priority=None  v=0 V  v_nominal_specify=off  v_nominal_value=1  v_nominal_unit=V  i_L_specify=off  i_L_priority=High  i_L=0 A  i_L_nominal_specify=off  i_L_nominal_value=1  i_L_nominal_unit=A
  Inductor2 : fl_lib/Electrical/Electrical Elements/Inductor  l=1e-6 H  r=0 Ohm  g=1e-9 1/Ohm  i_specify=off  i_priority=None  i=0 A  i_nominal_specify=off  i_nominal_value=1  i_nominal_unit=A  v_specify=off  v_priority=None  v=0 V  v_nominal_specify=off  v_nominal_value=1  v_nominal_unit=V  i_L_specify=off  i_L_priority=High  i_L=0 A  i_L_nominal_specify=off  i_L_nominal_value=1  i_L_nominal_unit=A
  threephase inductor : threephase_inductor_lib/threephase inductor  Lp=param.inv.hw.LFi H  L0=param.inv.hw.LFi_cm H  Rp=param.inv.hw.RLFi Ohm  R0=param.inv.hw.RLFi_cm Ohm  Lls=5e-6 H  uu_1_specify=off  uu_1_priority=None  uu_1=0 V  uu_1_nominal_specify=off  uu_1_nominal_value=1  uu_1_nominal_unit=V  uv_1_specify=off  uv_1_priority=None  uv_1=0 V  uv_1_nominal_specify=off  uv_1_nominal_value=1  uv_1_nominal_unit=V  uw_1_specify=off  uw_1_priority=None  uw_1=0 V  uw_1_nominal_specify=off  uw_1_nominal_value=1  uw_1_nominal_unit=V  uu_2_specify=off  uu_2_priority=None  uu_2=0 V  uu_2_nominal_specify=off  uu_2_nominal_value=1  uu_2_nominal_unit=V  uv_2_specify=off  uv_2_priority=None  uv_2=0 V  uv_2_nominal_specify=off  uv_2_nominal_value=1  uv_2_nominal_unit=V  uw_2_specify=off  uw_2_priority=None  uw_2=0 V  uw_2_nominal_specify=off  uw_2_nominal_value=1  uw_2_nominal_unit=V  iu_specify=off  iu_priority=None  iu=0 A  iu_nominal_specify=off  iu_nominal_value=1  iu_nominal_unit=A  iv_specify=off  iv_priority=None  iv=0 A  iv_nominal_specify=off  iv_nominal_value=1  iv_nominal_unit=A  iw_specify=off  iw_priority=None  iw=0 A  iw_nominal_specify=off  iw_nominal_value=1  iw_nominal_unit=A
  threephase_vi_measures_stack : Subsystem
  us_u : PMIOPort  Side=Left
  uu : PMIOPort  Port=2  Side=Right
  us_v : PMIOPort  Port=3  Side=Left
  uv : PMIOPort  Port=4  Side=Right
  us_w : PMIOPort  Port=5  Side=Left
  uw : PMIOPort  Port=6  Side=Right
  connections:
  threephase_vi_measures_stack/LConn1 -- us_u/RConn1
  threephase_vi_measures_stack/LConn2 -- us_v/RConn1
  threephase_vi_measures_stack/LConn3 -- us_w/RConn1
  threephase inductor/LConn1 -- threephase_vi_measures_stack/RConn1
  threephase inductor/LConn2 -- threephase_vi_measures_stack/RConn2
  threephase inductor/LConn3 -- threephase_vi_measures_stack/RConn3
  threephase inductor/RConn1 -- Inductor/LConn1
  threephase inductor/RConn2 -- Inductor1/LConn1
  threephase inductor/RConn3 -- Inductor2/LConn1
  Inductor/RConn1 -- uu/RConn1
  Inductor1/RConn1 -- uv/RConn1
  Inductor2/RConn1 -- uw/RConn1

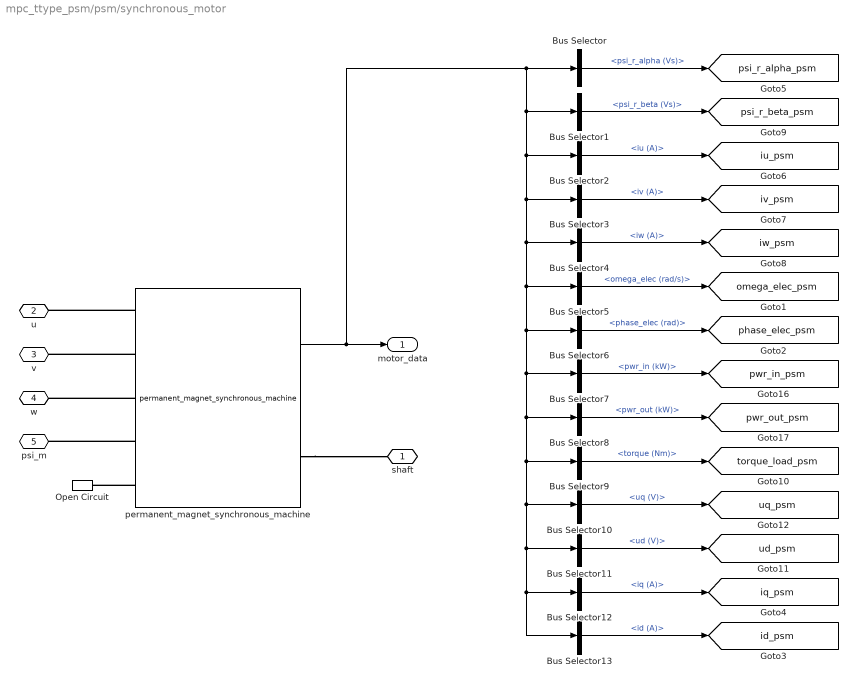
== system mpc_ttype_psm/psm/synchronous_motor ==
  Bus Selector : BusSelector  OutputSignals=psi_r_alpha (Vs)
  Bus Selector1 : BusSelector  OutputSignals=psi_r_beta (Vs)
  Bus Selector10 : BusSelector  OutputSignals=uq (V)
  Bus Selector11 : BusSelector  OutputSignals=ud (V)
  Bus Selector12 : BusSelector  OutputSignals=iq (A)
  Bus Selector13 : BusSelector  OutputSignals=id (A)
  Bus Selector2 : BusSelector  OutputSignals=iu (A)
  Bus Selector3 : BusSelector  OutputSignals=iv (A)
  Bus Selector4 : BusSelector  OutputSignals=iw (A)
  Bus Selector5 : BusSelector  OutputSignals=omega_elec (rad/s)
  Bus Selector6 : BusSelector  OutputSignals=phase_elec (rad)
  Bus Selector7 : BusSelector  OutputSignals=pwr_in (kW)
  Bus Selector8 : BusSelector  OutputSignals=pwr_out (kW)
  Bus Selector9 : BusSelector  OutputSignals=torque (Nm)
  Open Circuit : fl_lib/Electrical/Electrical Elements/Open Circuit  v_specify=off  v_priority=None  v=0 V  v_nominal_specify=off  v_nominal_value=1  v_nominal_unit=V
  permanent_magnet_synchronous_machine : permanent_magnet_synchronous_machine/permanent_magnet_synchronous_machine  pp=param.psm.machine.number_poles  psi_m=param.psm.machine.psi_m  Lmu=param.psm.machine.Lmu  La=param.psm.machine.La_m  Lb=param.psm.machine.Lb_m  Rs=param.psm.machine.Rs_m  Jm=param.psm.machine.Jm_m  b_linear=param.psm.machine.load_friction_m  b_quadratic=0  h5_percent=0  h7_percent=0  psi_r_u_init=param.psm.machine.psi_m  psi_r_v_init=-param.psm.machine.psi_m/2  psi_r_w_init=-param.psm.machine.psi_m/2  omega_init=0  phase_init=0
  shaft : PMIOPort  Side=Right
  u : PMIOPort  Port=2  Side=Left
  v : PMIOPort  Port=3  Side=Left
  w : PMIOPort  Port=4  Side=Left
  psi_m : PMIOPort  Port=5  Side=Left
  motor_data : Outport
  tag scope: id_psm=global, iq_psm=global, iu_psm=global, iv_psm=global, iw_psm=global, omega_elec_psm=global, phase_elec_psm=global, psi_r_alpha_psm=global, psi_r_beta_psm=global, pwr_in_psm=global, pwr_out_psm=global, torque_load_psm=global, ud_psm=global, uq_psm=global
  wires:
  permanent_magnet_synchronous_machine/1 -> Bus Selector8/1, Bus Selector10/1, Bus Selector11/1, Bus Selector12/1, Bus Selector13/1, Bus Selector9/1, Bus Selector7/1, Bus Selector6/1, Bus Selector5/1, Bus Selector4/1, Bus Selector3/1, Bus Selector2/1, Bus Selector1/1, Bus Selector/1, motor_data/1
  Bus Selector/1 -> [psi_r_alpha_psm]  "<psi_r_alpha (Vs)>"
  Bus Selector1/1 -> [psi_r_beta_psm]  "<psi_r_beta (Vs)>"
  Bus Selector2/1 -> [iu_psm]  "<iu (A)>"
  Bus Selector3/1 -> [iv_psm]  "<iv (A)>"
  Bus Selector4/1 -> [iw_psm]  "<iw (A)>"
  Bus Selector5/1 -> [omega_elec_psm]  "<omega_elec (rad/s)>"
  Bus Selector6/1 -> [phase_elec_psm]  "<phase_elec (rad)>"
  Bus Selector7/1 -> [pwr_in_psm]  "<pwr_in (kW)>"
  Bus Selector8/1 -> [pwr_out_psm]  "<pwr_out (kW)>"
  Bus Selector9/1 -> [torque_load_psm]  "<torque (Nm)>"
  Bus Selector10/1 -> [uq_psm]  "<uq (V)>"
  Bus Selector11/1 -> [ud_psm]  "<ud (V)>"
  Bus Selector12/1 -> [iq_psm]  "<iq (A)>"
  Bus Selector13/1 -> [id_psm]  "<id (A)>"
  connections:
  permanent_magnet_synchronous_machine/RConn1 -- shaft/RConn1
  permanent_magnet_synchronous_machine/LConn1 -- u/RConn1
  permanent_magnet_synchronous_machine/LConn2 -- v/RConn1
  permanent_magnet_synchronous_machine/LConn3 -- w/RConn1
  permanent_magnet_synchronous_machine/LConn4 -- psi_m/RConn1
  permanent_magnet_synchronous_machine/LConn5 -- Open Circuit/LConn1

== system mpc_ttype_psm/scopes/scopes_for_igbt_based_inverter ==
  Bus Creator1 : BusCreator  Inputs=2
  Bus Creator2 : BusCreator  Inputs=2
  Bus Creator6 : BusCreator  Inputs=2
  diode power losses INV Q1 : Scope  NumInputPorts=2
      settings: SampleTime=param.glb_time.tc  ActiveDisplayYMinimum=-1.5240099779957812  ActiveDisplayYMaximum=13.716019351034738  DataLoggingVariableName=ScopeData4
  igbt power losses INV Q1 : Scope  NumInputPorts=4
      settings: SampleTime=param.glb_time.tc  ActiveDisplayYMinimum=-146.40069949224531  ActiveDisplayYMaximum=1321.3065614948737  DataLoggingVariableName=ScopeData16
  igbt power losses INV Q2 : Scope  NumInputPorts=4
      settings: SampleTime=param.glb_time.tc  ActiveDisplayYMinimum=-59.27589767770079  ActiveDisplayYMaximum=564.40900084144926
  wires:
  [diode_JH_temp_invQ1] -> Bus Creator6/1  "diode_JH_temp_invQ1"
  [diode_ploss_invQ1] -> diode power losses INV Q1/1  "diode_ploss_invQ1"
  Bus Creator2/1 -> igbt power losses INV Q1/4
  [diode_HA_temp_invQ1] -> Bus Creator6/2  "diode_HA_temp_invQ1"
  [igbt_current_invQ1] -> igbt power losses INV Q1/2  "igbt_current_invQ1"
  [igbt_HA_temp_invQ1] -> Bus Creator2/2  "igbt_HA_temp_invQ1"
  Bus Creator1/1 -> igbt power losses INV Q2/4
  [igbt_voltage_invQ1] -> igbt power losses INV Q1/3  "igbt_voltage_invQ1"
  [igbt_JH_temp_invQ2] -> Bus Creator1/1  "igbt_JH_temp_invQ2"
  [igbt_current_invQ2] -> igbt power losses INV Q2/2  "igbt_current_invQ2"
  [igbt_ploss_invQ1] -> igbt power losses INV Q1/1  "igbt_ploss_invQ1"
  [igbt_HA_temp_invQ2] -> Bus Creator1/2  "igbt_HA_temp_invQ2"
  [igbt_JH_temp_invQ1] -> Bus Creator2/1  "igbt_JH_temp_invQ1"
  [igbt_ploss_invQ2] -> igbt power losses INV Q2/1  "igbt_ploss_invQ2"
  [igbt_voltage_invQ2] -> igbt power losses INV Q2/3  "igbt_voltage_invQ2"
  Bus Creator6/1 -> diode power losses INV Q1/2

== system mpc_ttype_psm/scopes/scopes_for_mosfet_based_inverter ==
  Bus Creator8 : BusCreator  Inputs=2
  Bus Creator9 : BusCreator  Inputs=2
  mosfet power losses INV Q1 : Scope  NumInputPorts=4
      settings: SampleTime=param.glb_time.tc  ActiveDisplayYMinimum=-32.258190719935513  ActiveDisplayYMaximum=388.05311151106906  DataLoggingVariableName=ScopeData28
  mosfet power losses INV Q2 : Scope  NumInputPorts=4
      settings: SampleTime=param.glb_time.tc  ActiveDisplayYMinimum=-60.051099059926763  ActiveDisplayYMaximum=540.45256909803  DataLoggingVariableName=ScopeData29
  wires:
  [mosfet_JH_temp_invQ1] -> Bus Creator8/1  "mosfet_JH_temp_invQ1"
  Bus Creator9/1 -> mosfet power losses INV Q2/4
  [mosfet_HA_temp_invQ2] -> Bus Creator9/2  "mosfet_HA_temp_invQ2"
  [mosfet_HA_temp_invQ1] -> Bus Creator8/2  "mosfet_HA_temp_invQ1"
  [mosfet_ploss_invQ2] -> mosfet power losses INV Q2/1  "mosfet_ploss_invQ2"
  [mosfet_JH_temp_invQ2] -> Bus Creator9/1  "mosfet_JH_temp_invQ2"
  [mosfet_current_invQ2] -> mosfet power losses INV Q2/3  "mosfet_current_invQ2"
  [mosfet_ploss_invQ1] -> mosfet power losses INV Q1/1  "mosfet_ploss_invQ1"
  [mosfet_voltage_invQ2] -> mosfet power losses INV Q2/2  "mosfet_voltage_invQ2"
  [mosfet_current_invQ1] -> mosfet power losses INV Q1/3  "mosfet_current_invQ1"
  Bus Creator8/1 -> mosfet power losses INV Q1/4
  [mosfet_voltage_invQ1] -> mosfet power losses INV Q1/2  "mosfet_voltage_invQ1"

== system mpc_ttype_psm/inv_psm_mod1/inverter/deadtime_generator_for_ttype ==
  gate_cmds_in : Inport
  Bus Creator : BusCreator  Inputs=3
  dead_time_generator_cmos_simulink_phu : Subsystem  mask{ts=param.glb_time.tc, positive_voltage_rail=15, dead_time=param.glb_time.dead_time_INV}
      mask prompts: ts "PT1 tau [s]"; positive_voltage_rail "Positive Voltage Rail [V]"; dead_time "DeadTime [s]"
  dead_time_generator_cmos_simulink_phv : Subsystem  mask{ts=param.glb_time.tc, positive_voltage_rail=15, dead_time=param.glb_time.dead_time_INV}
      mask prompts: ts "PT1 tau [s]"; positive_voltage_rail "Positive Voltage Rail [V]"; dead_time "DeadTime [s]"
  dead_time_generator_cmos_simulink_phw : Subsystem  mask{ts=param.glb_time.tc, positive_voltage_rail=15, dead_time=param.glb_time.dead_time_INV}
      mask prompts: ts "PT1 tau [s]"; positive_voltage_rail "Positive Voltage Rail [V]"; dead_time "DeadTime [s]"
  gate_cmds_out : Outport
  wires:
  Bus Creator/1 -> gate_cmds_out/1  "gate_cmds"
  dead_time_generator_cmos_simulink_phu/1(cmd_gates) -> Bus Creator/1  "gate_cmds_phu"
  gate_cmds_in/1 -> dead_time_generator_cmos_simulink_phu/1(gate_commands), dead_time_generator_cmos_simulink_phw/1(gate_commands), dead_time_generator_cmos_simulink_phv/1(gate_commands)
  dead_time_generator_cmos_simulink_phw/1(cmd_gates) -> Bus Creator/3  "gate_cmds_phw"
  dead_time_generator_cmos_simulink_phv/1(cmd_gates) -> Bus Creator/2  "gate_cmds_phv"

== system mpc_ttype_psm/inv_psm_mod1/inverter/timer ==
  time_source : Inport
  Constant1 : Constant  Value=double_sampling
  Constant2 : Constant  Value=0
  Constant8 : Constant  Value=tc
  Constant9 : Constant  Value=f
  MATLAB Function : MATLAB Function  TreatAsAtomicUnit=on  SystemSampleTime=tc
  MATLAB Function1 : single_phase_pwm_modulator/Single phase two level PWM generator with global TRGO/MATLAB Function1  SystemSampleTime=tc  VariantActivationTime=update diagram  EmptyChoice=off  PassThrough=off  PassThroughVariantControl=(default)  EmptyChoiceVariantControl=(default)  AllowFlexibleInterface=on  Latency=0  AutoFrameSizeCalculation=off
  period : Constant  Value=1/f
  TRGO : Outport
  wires:
  Constant1/1 -> MATLAB Function1/4
  time_source/1 -> MATLAB Function/1(t)
  Constant9/1 -> MATLAB Function1/2
  Constant8/1 -> MATLAB Function1/1
  MATLAB Function1/1 -> TRGO/1
  MATLAB Function/1(y) -> MATLAB Function1/3
  Constant2/1 -> MATLAB Function/2(phase)
  period/1 -> MATLAB Function/3(period)
